simulink model "Task4_Simscape_model"  (R2026a)
settings: Solver=FixedStepAuto  StopTime=8  FixedStep=0.001
model workspace (MATLAB code in the model file):
  | clear; clc; close all;
values from neighbouring files (symbols this model uses):
  A0 = 0.310447780017169    (= 0.310447780017)    [Parameters.m]    (also in Parameters_optimization.m)
  B10 = -0.192075602039053    (= -0.192075602039)    [Parameters.m]    (also in Parameters_optimization.m)
  B20 = -0.011912003704451    (= -0.0119120037045)    [Parameters.m]    (also in Parameters_optimization.m)
  black = partTemplate    [Parameters.m]    (also in Parameters_optimization.m = struct)
  blueBlock = partTemplate    [Parameters.m]    (also in Parameters_optimization.m = struct)
  cyan = partTemplate    [Parameters.m]    (also in Parameters_optimization.m = struct)
  g = 9.81    [Parameters.m]    (also in Parameters_optimization.m)
  G0 = -1.061422531644424    (= -1.06142253164)    [Parameters.m]    (also in Parameters_optimization.m)
  greenBeam = partTemplate    [Parameters.m]    (also in Parameters_optimization.m = struct)
  greenBlock = partTemplate    [Parameters.m]    (also in Parameters_optimization.m = struct)
  grey = partTemplate    [Parameters.m]    (also in Parameters_optimization.m = struct)
  H0 = -0.357470264672538    (= -0.357470264673)    [Parameters.m]    (also in Parameters_optimization.m)
  I0 = -1.033155420835947    (= -1.03315542084)    [Parameters.m]    (also in Parameters_optimization.m)
  JM = 0.002    [Parameters.m]    (also in Parameters_optimization.m)
  LB1 = 0.8    [Parameters.m]    (also in Parameters_optimization.m)
  LB2 = 0.3    [Parameters.m]    (also in Parameters_optimization.m)
  LB3 = 0.24    [Parameters.m]    (also in Parameters_optimization.m)
  Lblack1 = 0.2    [Parameters.m]    (also in Parameters_optimization.m)
  LC1 = 0.4    [Parameters.m]    (also in Parameters_optimization.m)
  LC2 = 0.225    [Parameters.m]    (also in Parameters_optimization.m)
  LG1 = 0.3    [Parameters.m]    (also in Parameters_optimization.m)
  LG2 = 0.8    [Parameters.m]    (also in Parameters_optimization.m)
  Lgrey1 = 1.175    [Parameters.m]    (also in Parameters_optimization.m)
  lightBlue = partTemplate    [Parameters.m]    (also in Parameters_optimization.m = struct)
  LLB1 = 0.248    [Parameters.m]    (also in Parameters_optimization.m)
  LLB2 = 0.235    [Parameters.m]    (also in Parameters_optimization.m)
  LR1 = 1.05    [Parameters.m]    (also in Parameters_optimization.m)
  LW1 = 1.05    [Parameters.m]    (also in Parameters_optimization.m)
  nA = 200    [Parameters.m]    (also in Parameters_optimization.m = 100)
  nB1 = 200    [Parameters.m]    (also in Parameters_optimization.m = 100)
  nB2 = 200    [Parameters.m]    (also in Parameters_optimization.m)
  nG = 20    [Parameters.m]    (also in Parameters_optimization.m)
  nH = 100    [Parameters.m]    (also in Parameters_optimization.m = 50)
  nI = 20    [Parameters.m]    (also in Parameters_optimization.m)
  red = partTemplate    [Parameters.m]    (also in Parameters_optimization.m = struct)
  trajCoeff = coeff    [Parameters.m]    (also in Parameters_optimization.m = [2000 500 1600; Path_Planning_Robot.m)
  trajTime = t    [Parameters.m]    (also in Parameters_optimization.m = [0 2 4 6 8]; Path_Planning_Robot.m)
  w = 0.1    [Parameters.m]    (also in Parameters_optimization.m)
  white = partTemplate    [Parameters.m]    (also in Parameters_optimization.m = struct)
undefined symbols (not defined in the file or in its folder): X, Y, Z
libraries: sm_lib x152, nesl_utility x69, simulink x1
(part 2 of 5)

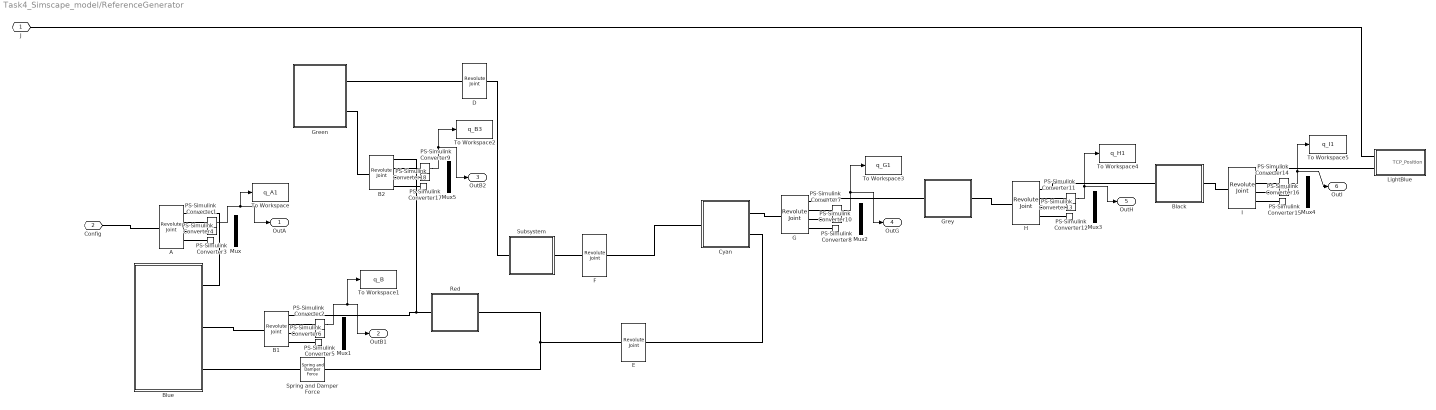
== system Task4_Simscape_model/ReferenceGenerator ==
  A : sm_lib/Joints/Revolute Joint  JointMode=Normal  CompositeWrenchDir=FollowerOnBase  CompositeWrenchFrame=BaseFrame  SenseConstraintForce=off  SenseConstraintTorque=off  SenseTotalForce=off  SenseTotalTorque=off  PositionTargetSpecify=off  PositionTargetPriority=High  PositionTargetValue=0  PositionTargetValueUnits=deg  VelocityTargetSpecify=off  VelocityTargetPriority=High  VelocityTargetValue=0  VelocityTargetValueUnits=deg/s  EquilibriumPosition=0  EquilibriumPositionUnits=deg  SpringStiffness=0  SpringStiffnessUnits=N*m/deg  DampingCoefficient=0  DampingCoefficientUnits=N*m/(deg/s)  LowerLimitSpecify=off  LowerLimitBound=-90  LowerLimitBoundUnits=deg  LowerLimitStiffness=1e4  LowerLimitStiffnessUnits=N*m/deg  LowerLimitDamping=10  LowerLimitDampingUnits=N*m/(deg/s)  LowerLimitTransitionRegionWidth=0.1  LowerLimitTransitionRegionWidthUnits=deg  UpperLimitSpecify=off  UpperLimitBound=90  UpperLimitBoundUnits=deg  UpperLimitStiffness=1e4  UpperLimitStiffnessUnits=N*m/deg  UpperLimitDamping=10  UpperLimitDampingUnits=N*m/(deg/s)  UpperLimitTransitionRegionWidth=0.1  UpperLimitTransitionRegionWidthUnits=deg  TorqueActuationMode=NoTorque  MotionActuationMode=ComputedMotion  SensePosition=on  SenseVelocity=on  SenseAcceleration=on  SenseTorqueForce=off  SenseLowerLimitTorqueForce=off  SenseUpperLimitTorqueForce=off
  B1 : sm_lib/Joints/Revolute Joint  JointMode=Normal  CompositeWrenchDir=FollowerOnBase  CompositeWrenchFrame=BaseFrame  SenseConstraintForce=off  SenseConstraintTorque=off  SenseTotalForce=off  SenseTotalTorque=off  PositionTargetSpecify=off  PositionTargetPriority=High  PositionTargetValue=0  PositionTargetValueUnits=deg  VelocityTargetSpecify=off  VelocityTargetPriority=High  VelocityTargetValue=0  VelocityTargetValueUnits=deg/s  EquilibriumPosition=0  EquilibriumPositionUnits=deg  SpringStiffness=0  SpringStiffnessUnits=N*m/deg  DampingCoefficient=0  DampingCoefficientUnits=N*m/(deg/s)  LowerLimitSpecify=on  LowerLimitBound=-80  LowerLimitBoundUnits=deg  LowerLimitStiffness=1e6  LowerLimitStiffnessUnits=N*m/deg  LowerLimitDamping=1000  LowerLimitDampingUnits=N*m/(deg/s)  LowerLimitTransitionRegionWidth=0.1  LowerLimitTransitionRegionWidthUnits=deg  UpperLimitSpecify=on  UpperLimitBound=80  UpperLimitBoundUnits=deg  UpperLimitStiffness=1e6  UpperLimitStiffnessUnits=N*m/deg  UpperLimitDamping=1000  UpperLimitDampingUnits=N*m/(deg/s)  UpperLimitTransitionRegionWidth=0.1  UpperLimitTransitionRegionWidthUnits=deg  TorqueActuationMode=NoTorque  MotionActuationMode=ComputedMotion  SensePosition=on  SenseVelocity=on  SenseAcceleration=on  SenseTorqueForce=off  SenseLowerLimitTorqueForce=off  SenseUpperLimitTorqueForce=off
  B2 : sm_lib/Joints/Revolute Joint  JointMode=Normal  CompositeWrenchDir=FollowerOnBase  CompositeWrenchFrame=BaseFrame  SenseConstraintForce=off  SenseConstraintTorque=off  SenseTotalForce=off  SenseTotalTorque=off  PositionTargetSpecify=off  PositionTargetPriority=High  PositionTargetValue=0  PositionTargetValueUnits=deg  VelocityTargetSpecify=off  VelocityTargetPriority=High  VelocityTargetValue=0  VelocityTargetValueUnits=deg/s  EquilibriumPosition=0  EquilibriumPositionUnits=deg  SpringStiffness=0  SpringStiffnessUnits=N*m/deg  DampingCoefficient=0  DampingCoefficientUnits=N*m/(deg/s)  LowerLimitSpecify=off  LowerLimitBound=-90  LowerLimitBoundUnits=deg  LowerLimitStiffness=1e4  LowerLimitStiffnessUnits=N*m/deg  LowerLimitDamping=10  LowerLimitDampingUnits=N*m/(deg/s)  LowerLimitTransitionRegionWidth=0.1  LowerLimitTransitionRegionWidthUnits=deg  UpperLimitSpecify=off  UpperLimitBound=90  UpperLimitBoundUnits=deg  UpperLimitStiffness=1e4  UpperLimitStiffnessUnits=N*m/deg  UpperLimitDamping=10  UpperLimitDampingUnits=N*m/(deg/s)  UpperLimitTransitionRegionWidth=0.1  UpperLimitTransitionRegionWidthUnits=deg  TorqueActuationMode=NoTorque  MotionActuationMode=ComputedMotion  SensePosition=on  SenseVelocity=on  SenseAcceleration=on  SenseTorqueForce=off  SenseLowerLimitTorqueForce=off  SenseUpperLimitTorqueForce=off
  Black : Subsystem
  Blue : Subsystem
  Cyan : Subsystem
  D : sm_lib/Joints/Revolute Joint  JointMode=Normal  CompositeWrenchDir=FollowerOnBase  CompositeWrenchFrame=BaseFrame  SenseConstraintForce=off  SenseConstraintTorque=off  SenseTotalForce=off  SenseTotalTorque=off  PositionTargetSpecify=off  PositionTargetPriority=High  PositionTargetValue=0  PositionTargetValueUnits=deg  VelocityTargetSpecify=off  VelocityTargetPriority=High  VelocityTargetValue=0  VelocityTargetValueUnits=deg/s  EquilibriumPosition=0  EquilibriumPositionUnits=deg  SpringStiffness=0  SpringStiffnessUnits=N*m/deg  DampingCoefficient=0  DampingCoefficientUnits=N*m/(deg/s)  LowerLimitSpecify=off  LowerLimitBound=-90  LowerLimitBoundUnits=deg  LowerLimitStiffness=1e4  LowerLimitStiffnessUnits=N*m/deg  LowerLimitDamping=10  LowerLimitDampingUnits=N*m/(deg/s)  LowerLimitTransitionRegionWidth=0.1  LowerLimitTransitionRegionWidthUnits=deg  UpperLimitSpecify=off  UpperLimitBound=90  UpperLimitBoundUnits=deg  UpperLimitStiffness=1e4  UpperLimitStiffnessUnits=N*m/deg  UpperLimitDamping=10  UpperLimitDampingUnits=N*m/(deg/s)  UpperLimitTransitionRegionWidth=0.1  UpperLimitTransitionRegionWidthUnits=deg  TorqueActuationMode=NoTorque  MotionActuationMode=ComputedMotion  SensePosition=off  SenseVelocity=off  SenseAcceleration=off  SenseTorqueForce=off  SenseLowerLimitTorqueForce=off  SenseUpperLimitTorqueForce=off
  E : sm_lib/Joints/Revolute Joint  JointMode=Normal  CompositeWrenchDir=FollowerOnBase  CompositeWrenchFrame=BaseFrame  SenseConstraintForce=off  SenseConstraintTorque=off  SenseTotalForce=off  SenseTotalTorque=off  PositionTargetSpecify=off  PositionTargetPriority=High  PositionTargetValue=0  PositionTargetValueUnits=deg  VelocityTargetSpecify=off  VelocityTargetPriority=High  VelocityTargetValue=0  VelocityTargetValueUnits=deg/s  EquilibriumPosition=0  EquilibriumPositionUnits=deg  SpringStiffness=0  SpringStiffnessUnits=N*m/deg  DampingCoefficient=0  DampingCoefficientUnits=N*m/(deg/s)  LowerLimitSpecify=on  LowerLimitBound=-80  LowerLimitBoundUnits=deg  LowerLimitStiffness=1e6  LowerLimitStiffnessUnits=N*m/deg  LowerLimitDamping=100000  LowerLimitDampingUnits=N*m/(deg/s)  LowerLimitTransitionRegionWidth=0.1  LowerLimitTransitionRegionWidthUnits=deg  UpperLimitSpecify=on  UpperLimitBound=80  UpperLimitBoundUnits=deg  UpperLimitStiffness=1e6  UpperLimitStiffnessUnits=N*m/deg  UpperLimitDamping=100000  UpperLimitDampingUnits=N*m/(deg/s)  UpperLimitTransitionRegionWidth=0.1  UpperLimitTransitionRegionWidthUnits=deg  TorqueActuationMode=NoTorque  MotionActuationMode=ComputedMotion  SensePosition=off  SenseVelocity=off  SenseAcceleration=off  SenseTorqueForce=off  SenseLowerLimitTorqueForce=off  SenseUpperLimitTorqueForce=off
  F : sm_lib/Joints/Revolute Joint  JointMode=Normal  CompositeWrenchDir=FollowerOnBase  CompositeWrenchFrame=BaseFrame  SenseConstraintForce=off  SenseConstraintTorque=off  SenseTotalForce=off  SenseTotalTorque=off  PositionTargetSpecify=off  PositionTargetPriority=High  PositionTargetValue=0  PositionTargetValueUnits=deg  VelocityTargetSpecify=off  VelocityTargetPriority=High  VelocityTargetValue=0  VelocityTargetValueUnits=deg/s  EquilibriumPosition=0  EquilibriumPositionUnits=deg  SpringStiffness=0  SpringStiffnessUnits=N*m/deg  DampingCoefficient=0  DampingCoefficientUnits=N*m/(deg/s)  LowerLimitSpecify=off  LowerLimitBound=-90  LowerLimitBoundUnits=deg  LowerLimitStiffness=1e4  LowerLimitStiffnessUnits=N*m/deg  LowerLimitDamping=10  LowerLimitDampingUnits=N*m/(deg/s)  LowerLimitTransitionRegionWidth=0.1  LowerLimitTransitionRegionWidthUnits=deg  UpperLimitSpecify=off  UpperLimitBound=90  UpperLimitBoundUnits=deg  UpperLimitStiffness=1e4  UpperLimitStiffnessUnits=N*m/deg  UpperLimitDamping=10  UpperLimitDampingUnits=N*m/(deg/s)  UpperLimitTransitionRegionWidth=0.1  UpperLimitTransitionRegionWidthUnits=deg  TorqueActuationMode=NoTorque  MotionActuationMode=ComputedMotion  SensePosition=off  SenseVelocity=off  SenseAcceleration=off  SenseTorqueForce=off  SenseLowerLimitTorqueForce=off  SenseUpperLimitTorqueForce=off
  G : sm_lib/Joints/Revolute Joint  JointMode=Normal  CompositeWrenchDir=FollowerOnBase  CompositeWrenchFrame=BaseFrame  SenseConstraintForce=off  SenseConstraintTorque=off  SenseTotalForce=off  SenseTotalTorque=off  PositionTargetSpecify=off  PositionTargetPriority=High  PositionTargetValue=0  PositionTargetValueUnits=deg  VelocityTargetSpecify=off  VelocityTargetPriority=High  VelocityTargetValue=0  VelocityTargetValueUnits=deg/s  EquilibriumPosition=0  EquilibriumPositionUnits=deg  SpringStiffness=0  SpringStiffnessUnits=N*m/deg  DampingCoefficient=0  DampingCoefficientUnits=N*m/(deg/s)  LowerLimitSpecify=off  LowerLimitBound=-90  LowerLimitBoundUnits=deg  LowerLimitStiffness=1e4  LowerLimitStiffnessUnits=N*m/deg  LowerLimitDamping=10  LowerLimitDampingUnits=N*m/(deg/s)  LowerLimitTransitionRegionWidth=0.1  LowerLimitTransitionRegionWidthUnits=deg  UpperLimitSpecify=off  UpperLimitBound=90  UpperLimitBoundUnits=deg  UpperLimitStiffness=1e4  UpperLimitStiffnessUnits=N*m/deg  UpperLimitDamping=10  UpperLimitDampingUnits=N*m/(deg/s)  UpperLimitTransitionRegionWidth=0.1  UpperLimitTransitionRegionWidthUnits=deg  TorqueActuationMode=NoTorque  MotionActuationMode=ComputedMotion  SensePosition=on  SenseVelocity=on  SenseAcceleration=on  SenseTorqueForce=off  SenseLowerLimitTorqueForce=off  SenseUpperLimitTorqueForce=off
  Green : Subsystem
  Grey : Subsystem
  H : sm_lib/Joints/Revolute Joint  JointMode=Normal  CompositeWrenchDir=FollowerOnBase  CompositeWrenchFrame=BaseFrame  SenseConstraintForce=off  SenseConstraintTorque=off  SenseTotalForce=off  SenseTotalTorque=off  PositionTargetSpecify=off  PositionTargetPriority=High  PositionTargetValue=0  PositionTargetValueUnits=deg  VelocityTargetSpecify=off  VelocityTargetPriority=High  VelocityTargetValue=0  VelocityTargetValueUnits=deg/s  EquilibriumPosition=0  EquilibriumPositionUnits=deg  SpringStiffness=0  SpringStiffnessUnits=N*m/deg  DampingCoefficient=0  DampingCoefficientUnits=N*m/(deg/s)  LowerLimitSpecify=on  LowerLimitBound=-90  LowerLimitBoundUnits=deg  LowerLimitStiffness=1e4  LowerLimitStiffnessUnits=N*m/deg  LowerLimitDamping=10  LowerLimitDampingUnits=N*m/(deg/s)  LowerLimitTransitionRegionWidth=0.1  LowerLimitTransitionRegionWidthUnits=deg  UpperLimitSpecify=on  UpperLimitBound=90  UpperLimitBoundUnits=deg  UpperLimitStiffness=1e4  UpperLimitStiffnessUnits=N*m/deg  UpperLimitDamping=10  UpperLimitDampingUnits=N*m/(deg/s)  UpperLimitTransitionRegionWidth=0.1  UpperLimitTransitionRegionWidthUnits=deg  TorqueActuationMode=NoTorque  MotionActuationMode=ComputedMotion  SensePosition=on  SenseVelocity=on  SenseAcceleration=on  SenseTorqueForce=off  SenseLowerLimitTorqueForce=off  SenseUpperLimitTorqueForce=off
  I : sm_lib/Joints/Revolute Joint  JointMode=Normal  CompositeWrenchDir=FollowerOnBase  CompositeWrenchFrame=BaseFrame  SenseConstraintForce=off  SenseConstraintTorque=off  SenseTotalForce=off  SenseTotalTorque=off  PositionTargetSpecify=off  PositionTargetPriority=High  PositionTargetValue=0  PositionTargetValueUnits=deg  VelocityTargetSpecify=off  VelocityTargetPriority=High  VelocityTargetValue=0  VelocityTargetValueUnits=deg/s  EquilibriumPosition=0  EquilibriumPositionUnits=deg  SpringStiffness=0  SpringStiffnessUnits=N*m/deg  DampingCoefficient=0  DampingCoefficientUnits=N*m/(deg/s)  LowerLimitSpecify=off  LowerLimitBound=-90  LowerLimitBoundUnits=deg  LowerLimitStiffness=1e4  LowerLimitStiffnessUnits=N*m/deg  LowerLimitDamping=10  LowerLimitDampingUnits=N*m/(deg/s)  LowerLimitTransitionRegionWidth=0.1  LowerLimitTransitionRegionWidthUnits=deg  UpperLimitSpecify=off  UpperLimitBound=90  UpperLimitBoundUnits=deg  UpperLimitStiffness=1e4  UpperLimitStiffnessUnits=N*m/deg  UpperLimitDamping=10  UpperLimitDampingUnits=N*m/(deg/s)  UpperLimitTransitionRegionWidth=0.1  UpperLimitTransitionRegionWidthUnits=deg  TorqueActuationMode=NoTorque  MotionActuationMode=ComputedMotion  SensePosition=on  SenseVelocity=on  SenseAcceleration=on  SenseTorqueForce=off  SenseLowerLimitTorqueForce=off  SenseUpperLimitTorqueForce=off
  LightBlue : Subsystem
  Mux{,1..5} (6 alike) : Mux  Inputs=3
  PS-Simulink Converter{1..18} (18 alike) : nesl_utility/PS-Simulink Converter  PhysicalDomain=network_engine_domain  SubClassName=ps_output  LeftPortType=input  RightPortType=output  PseudoPeriodic=off  Frequencies=[]  VectorFormat=inherit  Unit=inherit  AffineConversion=off
  Red : Subsystem
  Spring and Damper Force : sm_lib/Forces and Torques/Spring and Damper Force  NaturalLength=L0_spring  NaturalLengthUnits=m  SpringStiffness=k_spring  SpringStiffnessUnits=N/m  DampingCoefficient=0  DampingCoefficientUnits=N/(m/s)  SenseForce=off
  Subsystem : Subsystem
  To Workspace : ToWorkspace  VariableName=q_A1  SaveFormat=Timeseries  SampleTime=-1
  To Workspace1 : ToWorkspace  VariableName=q_B  SaveFormat=Timeseries  SampleTime=-1
  To Workspace2 : ToWorkspace  VariableName=q_B3  SaveFormat=Timeseries  SampleTime=-1
  To Workspace3 : ToWorkspace  VariableName=q_G1  SaveFormat=Timeseries  SampleTime=-1
  To Workspace4 : ToWorkspace  VariableName=q_H1  SaveFormat=Timeseries  SampleTime=-1
  To Workspace5 : ToWorkspace  VariableName=q_I1  SaveFormat=Timeseries  SampleTime=-1
  J : PMIOPort  Side=Left
  Config : PMIOPort  Port=2  Side=Left
  OutA : Outport
  OutB1 : Outport  Port=2
  OutB2 : Outport  Port=3
  OutG : Outport  Port=4
  OutH : Outport  Port=5
  OutI : Outport  Port=6
  wires:
  PS-Simulink Converter2/1 -> To Workspace1/1, OutB1/1
  PS-Simulink Converter1/1 -> To Workspace/1, OutA/1
  PS-Simulink Converter9/1 -> To Workspace2/1, OutB2/1
  PS-Simulink Converter7/1 -> To Workspace3/1, OutG/1
  PS-Simulink Converter11/1 -> To Workspace4/1, OutH/1
  PS-Simulink Converter14/1 -> To Workspace5/1, OutI/1
  connections:
  B2/RConn1 -- B1/RConn1 -- Red/RConn1
  LightBlue/LConn2 -- I/RConn1
  G/LConn1 -- Cyan/RConn1
  Spring and Damper Force/RConn1 -- Red/LConn1 -- E/LConn1
  Black/LConn1 -- H/RConn1
  F/LConn1 -- Subsystem/LConn1
  Spring and Damper Force/LConn1 -- Blue/RConn3
  Subsystem/RConn1 -- D/RConn1
  Green/RConn2 -- B2/LConn1
  I/LConn1 -- Black/RConn1
  A/LConn1 -- Config/RConn1
  Blue/RConn2 -- B1/LConn1
  H/LConn1 -- Grey/RConn1
  F/RConn1 -- Cyan/LConn1
  D/LConn1 -- Green/RConn1
  Grey/LConn1 -- G/RConn1
  Blue/RConn1 -- A/RConn1
  Cyan/RConn2 -- E/RConn1
  J/RConn1 -- LightBlue/LConn1
  PS-Simulink Converter1/LConn1 -- A/RConn2
  PS-Simulink Converter3/LConn1 -- A/RConn3
  PS-Simulink Converter4/LConn1 -- A/RConn4
  PS-Simulink Converter2/LConn1 -- B1/RConn2
  B1/RConn3 -- PS-Simulink Converter5/LConn1
  PS-Simulink Converter6/LConn1 -- B1/RConn4
  PS-Simulink Converter7/LConn1 -- G/RConn2
  G/RConn3 -- PS-Simulink Converter8/LConn1
  PS-Simulink Converter10/LConn1 -- G/RConn4
  PS-Simulink Converter11/LConn1 -- H/RConn2
  PS-Simulink Converter12/LConn1 -- H/RConn3
  PS-Simulink Converter13/LConn1 -- H/RConn4
  PS-Simulink Converter14/LConn1 -- I/RConn2
  PS-Simulink Converter15/LConn1 -- I/RConn3
  PS-Simulink Converter16/LConn1 -- I/RConn4
  PS-Simulink Converter9/LConn1 -- B2/RConn2
  PS-Simulink Converter17/LConn1 -- B2/RConn3
  PS-Simulink Converter18/LConn1 -- B2/RConn4

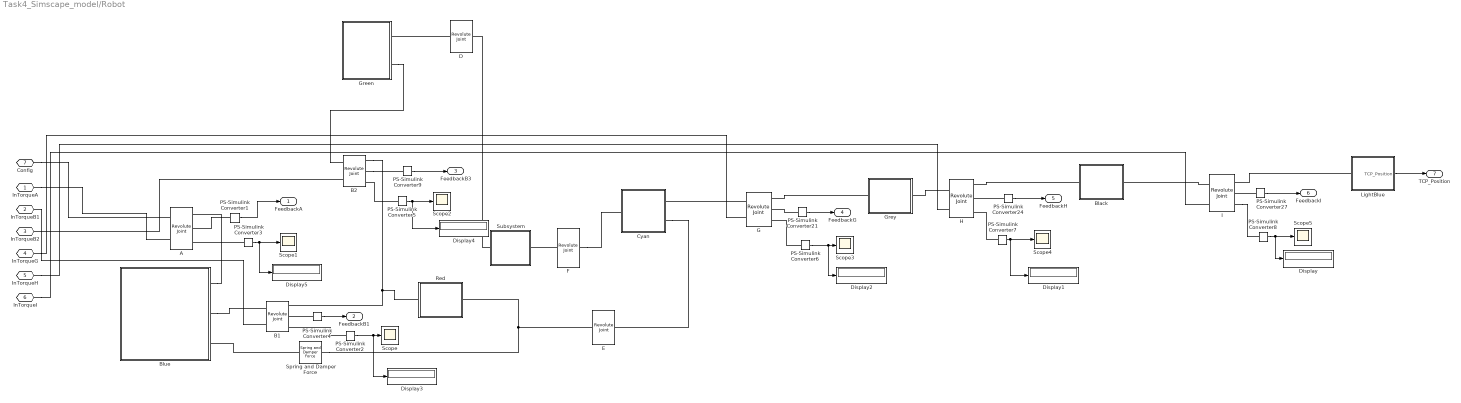
== system Task4_Simscape_model/Robot ==
  A : sm_lib/Joints/Revolute Joint  JointMode=Normal  CompositeWrenchDir=FollowerOnBase  CompositeWrenchFrame=BaseFrame  SenseConstraintForce=off  SenseConstraintTorque=off  SenseTotalForce=off  SenseTotalTorque=off  PositionTargetSpecify=on  PositionTargetPriority=High  PositionTargetValue=A0  PositionTargetValueUnits=rad  VelocityTargetSpecify=on  VelocityTargetPriority=High  VelocityTargetValue=0  VelocityTargetValueUnits=rad/s  EquilibriumPosition=0  EquilibriumPositionUnits=deg  SpringStiffness=0  SpringStiffnessUnits=N*m/deg  DampingCoefficient=0  DampingCoefficientUnits=N*m/(deg/s)  LowerLimitSpecify=off  LowerLimitBound=-90  LowerLimitBoundUnits=deg  LowerLimitStiffness=1e4  LowerLimitStiffnessUnits=N*m/deg  LowerLimitDamping=10  LowerLimitDampingUnits=N*m/(deg/s)  LowerLimitTransitionRegionWidth=0.1  LowerLimitTransitionRegionWidthUnits=deg  UpperLimitSpecify=off  UpperLimitBound=90  UpperLimitBoundUnits=deg  UpperLimitStiffness=1e4  UpperLimitStiffnessUnits=N*m/deg  UpperLimitDamping=10  UpperLimitDampingUnits=N*m/(deg/s)  UpperLimitTransitionRegionWidth=0.1  UpperLimitTransitionRegionWidthUnits=deg  TorqueActuationMode=InputTorque  MotionActuationMode=ComputedMotion  SensePosition=on  SenseVelocity=off  SenseAcceleration=off  SenseTorqueForce=on  SenseLowerLimitTorqueForce=off  SenseUpperLimitTorqueForce=off
  B1 : sm_lib/Joints/Revolute Joint  JointMode=Normal  CompositeWrenchDir=FollowerOnBase  CompositeWrenchFrame=BaseFrame  SenseConstraintForce=off  SenseConstraintTorque=off  SenseTotalForce=off  SenseTotalTorque=off  PositionTargetSpecify=on  PositionTargetPriority=High  PositionTargetValue=B10  PositionTargetValueUnits=rad  VelocityTargetSpecify=on  VelocityTargetPriority=High  VelocityTargetValue=0  VelocityTargetValueUnits=rad/s  EquilibriumPosition=0  EquilibriumPositionUnits=deg  SpringStiffness=0  SpringStiffnessUnits=N*m/deg  DampingCoefficient=0  DampingCoefficientUnits=N*m/(deg/s)  LowerLimitSpecify=on  LowerLimitBound=-80  LowerLimitBoundUnits=deg  LowerLimitStiffness=1000  LowerLimitStiffnessUnits=N*m/deg  LowerLimitDamping=1000  LowerLimitDampingUnits=N*m/(deg/s)  LowerLimitTransitionRegionWidth=0.1  LowerLimitTransitionRegionWidthUnits=deg  UpperLimitSpecify=on  UpperLimitBound=80  UpperLimitBoundUnits=deg  UpperLimitStiffness=1000  UpperLimitStiffnessUnits=N*m/deg  UpperLimitDamping=1000  UpperLimitDampingUnits=N*m/(deg/s)  UpperLimitTransitionRegionWidth=0.1  UpperLimitTransitionRegionWidthUnits=deg  TorqueActuationMode=InputTorque  MotionActuationMode=ComputedMotion  SensePosition=on  SenseVelocity=off  SenseAcceleration=off  SenseTorqueForce=on  SenseLowerLimitTorqueForce=off  SenseUpperLimitTorqueForce=off
  B2 : sm_lib/Joints/Revolute Joint  JointMode=Normal  CompositeWrenchDir=FollowerOnBase  CompositeWrenchFrame=BaseFrame  SenseConstraintForce=off  SenseConstraintTorque=off  SenseTotalForce=off  SenseTotalTorque=off  PositionTargetSpecify=on  PositionTargetPriority=High  PositionTargetValue=B20  PositionTargetValueUnits=rad  VelocityTargetSpecify=on  VelocityTargetPriority=High  VelocityTargetValue=0  VelocityTargetValueUnits=rad/s  EquilibriumPosition=0  EquilibriumPositionUnits=deg  SpringStiffness=0  SpringStiffnessUnits=N*m/deg  DampingCoefficient=0  DampingCoefficientUnits=N*m/(deg/s)  LowerLimitSpecify=off  LowerLimitBound=-90  LowerLimitBoundUnits=deg  LowerLimitStiffness=1e4  LowerLimitStiffnessUnits=N*m/deg  LowerLimitDamping=10  LowerLimitDampingUnits=N*m/(deg/s)  LowerLimitTransitionRegionWidth=0.1  LowerLimitTransitionRegionWidthUnits=deg  UpperLimitSpecify=off  UpperLimitBound=90  UpperLimitBoundUnits=deg  UpperLimitStiffness=1e4  UpperLimitStiffnessUnits=N*m/deg  UpperLimitDamping=10  UpperLimitDampingUnits=N*m/(deg/s)  UpperLimitTransitionRegionWidth=0.1  UpperLimitTransitionRegionWidthUnits=deg  TorqueActuationMode=InputTorque  MotionActuationMode=ComputedMotion  SensePosition=on  SenseVelocity=off  SenseAcceleration=off  SenseTorqueForce=on  SenseLowerLimitTorqueForce=off  SenseUpperLimitTorqueForce=off
  Black : Subsystem
  Blue : Subsystem
  Cyan : Subsystem
  D : sm_lib/Joints/Revolute Joint  JointMode=Normal  CompositeWrenchDir=FollowerOnBase  CompositeWrenchFrame=BaseFrame  SenseConstraintForce=off  SenseConstraintTorque=off  SenseTotalForce=off  SenseTotalTorque=off  PositionTargetSpecify=off  PositionTargetPriority=High  PositionTargetValue=0  PositionTargetValueUnits=deg  VelocityTargetSpecify=off  VelocityTargetPriority=High  VelocityTargetValue=0  VelocityTargetValueUnits=deg/s  EquilibriumPosition=0  EquilibriumPositionUnits=deg  SpringStiffness=0  SpringStiffnessUnits=N*m/deg  DampingCoefficient=0  DampingCoefficientUnits=N*m/(deg/s)  LowerLimitSpecify=off  LowerLimitBound=-90  LowerLimitBoundUnits=deg  LowerLimitStiffness=1e4  LowerLimitStiffnessUnits=N*m/deg  LowerLimitDamping=10  LowerLimitDampingUnits=N*m/(deg/s)  LowerLimitTransitionRegionWidth=0.1  LowerLimitTransitionRegionWidthUnits=deg  UpperLimitSpecify=off  UpperLimitBound=90  UpperLimitBoundUnits=deg  UpperLimitStiffness=1e4  UpperLimitStiffnessUnits=N*m/deg  UpperLimitDamping=10  UpperLimitDampingUnits=N*m/(deg/s)  UpperLimitTransitionRegionWidth=0.1  UpperLimitTransitionRegionWidthUnits=deg  TorqueActuationMode=NoTorque  MotionActuationMode=ComputedMotion  SensePosition=off  SenseVelocity=off  SenseAcceleration=off  SenseTorqueForce=off  SenseLowerLimitTorqueForce=off  SenseUpperLimitTorqueForce=off
  Display{,1..5} (6 alike) : Display
  E : sm_lib/Joints/Revolute Joint  JointMode=Normal  CompositeWrenchDir=FollowerOnBase  CompositeWrenchFrame=BaseFrame  SenseConstraintForce=off  SenseConstraintTorque=off  SenseTotalForce=off  SenseTotalTorque=off  PositionTargetSpecify=off  PositionTargetPriority=High  PositionTargetValue=0  PositionTargetValueUnits=deg  VelocityTargetSpecify=off  VelocityTargetPriority=High  VelocityTargetValue=0  VelocityTargetValueUnits=deg/s  EquilibriumPosition=0  EquilibriumPositionUnits=deg  SpringStiffness=0  SpringStiffnessUnits=N*m/deg  DampingCoefficient=0  DampingCoefficientUnits=N*m/(deg/s)  LowerLimitSpecify=on  LowerLimitBound=-80  LowerLimitBoundUnits=deg  LowerLimitStiffness=1e6  LowerLimitStiffnessUnits=N*m/deg  LowerLimitDamping=100000  LowerLimitDampingUnits=N*m/(deg/s)  LowerLimitTransitionRegionWidth=0.1  LowerLimitTransitionRegionWidthUnits=deg  UpperLimitSpecify=on  UpperLimitBound=80  UpperLimitBoundUnits=deg  UpperLimitStiffness=1e6  UpperLimitStiffnessUnits=N*m/deg  UpperLimitDamping=100000  UpperLimitDampingUnits=N*m/(deg/s)  UpperLimitTransitionRegionWidth=0.1  UpperLimitTransitionRegionWidthUnits=deg  TorqueActuationMode=NoTorque  MotionActuationMode=ComputedMotion  SensePosition=off  SenseVelocity=off  SenseAcceleration=off  SenseTorqueForce=off  SenseLowerLimitTorqueForce=off  SenseUpperLimitTorqueForce=off
  F : sm_lib/Joints/Revolute Joint  JointMode=Normal  CompositeWrenchDir=FollowerOnBase  CompositeWrenchFrame=BaseFrame  SenseConstraintForce=off  SenseConstraintTorque=off  SenseTotalForce=off  SenseTotalTorque=off  PositionTargetSpecify=off  PositionTargetPriority=High  PositionTargetValue=0  PositionTargetValueUnits=deg  VelocityTargetSpecify=off  VelocityTargetPriority=High  VelocityTargetValue=0  VelocityTargetValueUnits=deg/s  EquilibriumPosition=0  EquilibriumPositionUnits=deg  SpringStiffness=0  SpringStiffnessUnits=N*m/deg  DampingCoefficient=0  DampingCoefficientUnits=N*m/(deg/s)  LowerLimitSpecify=off  LowerLimitBound=-90  LowerLimitBoundUnits=deg  LowerLimitStiffness=1e4  LowerLimitStiffnessUnits=N*m/deg  LowerLimitDamping=10  LowerLimitDampingUnits=N*m/(deg/s)  LowerLimitTransitionRegionWidth=0.1  LowerLimitTransitionRegionWidthUnits=deg  UpperLimitSpecify=off  UpperLimitBound=90  UpperLimitBoundUnits=deg  UpperLimitStiffness=1e4  UpperLimitStiffnessUnits=N*m/deg  UpperLimitDamping=10  UpperLimitDampingUnits=N*m/(deg/s)  UpperLimitTransitionRegionWidth=0.1  UpperLimitTransitionRegionWidthUnits=deg  TorqueActuationMode=NoTorque  MotionActuationMode=ComputedMotion  SensePosition=off  SenseVelocity=off  SenseAcceleration=off  SenseTorqueForce=off  SenseLowerLimitTorqueForce=off  SenseUpperLimitTorqueForce=off
  G : sm_lib/Joints/Revolute Joint  JointMode=Normal  CompositeWrenchDir=FollowerOnBase  CompositeWrenchFrame=BaseFrame  SenseConstraintForce=off  SenseConstraintTorque=off  SenseTotalForce=off  SenseTotalTorque=off  PositionTargetSpecify=on  PositionTargetPriority=High  PositionTargetValue=G0  PositionTargetValueUnits=rad  VelocityTargetSpecify=on  VelocityTargetPriority=High  VelocityTargetValue=0  VelocityTargetValueUnits=rad/s  EquilibriumPosition=0  EquilibriumPositionUnits=deg  SpringStiffness=0  SpringStiffnessUnits=N*m/deg  DampingCoefficient=0  DampingCoefficientUnits=N*m/(deg/s)  LowerLimitSpecify=off  LowerLimitBound=-90  LowerLimitBoundUnits=deg  LowerLimitStiffness=1e4  LowerLimitStiffnessUnits=N*m/deg  LowerLimitDamping=10  LowerLimitDampingUnits=N*m/(deg/s)  LowerLimitTransitionRegionWidth=0.1  LowerLimitTransitionRegionWidthUnits=deg  UpperLimitSpecify=off  UpperLimitBound=90  UpperLimitBoundUnits=deg  UpperLimitStiffness=1e4  UpperLimitStiffnessUnits=N*m/deg  UpperLimitDamping=10  UpperLimitDampingUnits=N*m/(deg/s)  UpperLimitTransitionRegionWidth=0.1  UpperLimitTransitionRegionWidthUnits=deg  TorqueActuationMode=InputTorque  MotionActuationMode=ComputedMotion  SensePosition=on  SenseVelocity=off  SenseAcceleration=off  SenseTorqueForce=on  SenseLowerLimitTorqueForce=off  SenseUpperLimitTorqueForce=off
  Green : Subsystem
  Grey : Subsystem
  H : sm_lib/Joints/Revolute Joint  JointMode=Normal  CompositeWrenchDir=FollowerOnBase  CompositeWrenchFrame=BaseFrame  SenseConstraintForce=off  SenseConstraintTorque=off  SenseTotalForce=off  SenseTotalTorque=off  PositionTargetSpecify=on  PositionTargetPriority=High  PositionTargetValue=H0  PositionTargetValueUnits=rad  VelocityTargetSpecify=on  VelocityTargetPriority=High  VelocityTargetValue=0  VelocityTargetValueUnits=rad/s  EquilibriumPosition=0  EquilibriumPositionUnits=deg  SpringStiffness=0  SpringStiffnessUnits=N*m/deg  DampingCoefficient=0  DampingCoefficientUnits=N*m/(deg/s)  LowerLimitSpecify=off  LowerLimitBound=-90  LowerLimitBoundUnits=deg  LowerLimitStiffness=100  LowerLimitStiffnessUnits=N*m/deg  LowerLimitDamping=1000  LowerLimitDampingUnits=N*m/(deg/s)  LowerLimitTransitionRegionWidth=0.1  LowerLimitTransitionRegionWidthUnits=deg  UpperLimitSpecify=off  UpperLimitBound=90  UpperLimitBoundUnits=deg  UpperLimitStiffness=100  UpperLimitStiffnessUnits=N*m/deg  UpperLimitDamping=1000  UpperLimitDampingUnits=N*m/(deg/s)  UpperLimitTransitionRegionWidth=0.1  UpperLimitTransitionRegionWidthUnits=deg  TorqueActuationMode=InputTorque  MotionActuationMode=ComputedMotion  SensePosition=on  SenseVelocity=off  SenseAcceleration=off  SenseTorqueForce=on  SenseLowerLimitTorqueForce=off  SenseUpperLimitTorqueForce=off
  I : sm_lib/Joints/Revolute Joint  JointMode=Normal  CompositeWrenchDir=FollowerOnBase  CompositeWrenchFrame=BaseFrame  SenseConstraintForce=off  SenseConstraintTorque=off  SenseTotalForce=off  SenseTotalTorque=off  PositionTargetSpecify=on  PositionTargetPriority=High  PositionTargetValue=I0  PositionTargetValueUnits=rad  VelocityTargetSpecify=on  VelocityTargetPriority=High  VelocityTargetValue=0  VelocityTargetValueUnits=rad/s  EquilibriumPosition=0  EquilibriumPositionUnits=deg  SpringStiffness=0  SpringStiffnessUnits=N*m/deg  DampingCoefficient=0  DampingCoefficientUnits=N*m/(deg/s)  LowerLimitSpecify=on  LowerLimitBound=-90  LowerLimitBoundUnits=deg  LowerLimitStiffness=1e5  LowerLimitStiffnessUnits=N*m/deg  LowerLimitDamping=100  LowerLimitDampingUnits=N*m/(deg/s)  LowerLimitTransitionRegionWidth=0.1  LowerLimitTransitionRegionWidthUnits=deg  UpperLimitSpecify=on  UpperLimitBound=90  UpperLimitBoundUnits=deg  UpperLimitStiffness=1e5  UpperLimitStiffnessUnits=N*m/deg  UpperLimitDamping=100  UpperLimitDampingUnits=N*m/(deg/s)  UpperLimitTransitionRegionWidth=0.1  UpperLimitTransitionRegionWidthUnits=deg  TorqueActuationMode=InputTorque  MotionActuationMode=ComputedMotion  SensePosition=on  SenseVelocity=off  SenseAcceleration=off  SenseTorqueForce=on  SenseLowerLimitTorqueForce=off  SenseUpperLimitTorqueForce=off
  LightBlue : Subsystem
  PS-Simulink Converter{1..9,21,24,27} (12 alike) : nesl_utility/PS-Simulink Converter  PhysicalDomain=network_engine_domain  SubClassName=ps_output  LeftPortType=input  RightPortType=output  PseudoPeriodic=off  Frequencies=[]  VectorFormat=inherit  Unit=inherit  AffineConversion=off
  Red : Subsystem
  Scope{,1..5} (6 alike) : Scope
      Scope settings: ActiveDisplayYMinimum=-1183.9928415101156  ActiveDisplayYMaximum=-1183.9928415101133  DataLoggingVariableName=ScopeData10
      Scope1 settings: ActiveDisplayYMinimum=-1  ActiveDisplayYMaximum=1  DataLoggingVariableName=ScopeData11
      Scope2 settings: ActiveDisplayYMinimum=-1  ActiveDisplayYMaximum=1  DataLoggingVariableName=ScopeData12
      Scope3 settings: ActiveDisplayYMinimum=76.287342511896966  ActiveDisplayYMaximum=76.2873425118971  DataLoggingVariableName=ScopeData13
      Scope4 settings: ActiveDisplayYMinimum=-1  ActiveDisplayYMaximum=1  DataLoggingVariableName=ScopeData14
      Scope5 settings: ActiveDisplayYMinimum=-1  ActiveDisplayYMaximum=1  DataLoggingVariableName=ScopeData15
  Spring and Damper Force : sm_lib/Forces and Torques/Spring and Damper Force  NaturalLength=L0_spring  NaturalLengthUnits=m  SpringStiffness=k_spring  SpringStiffnessUnits=N/m  DampingCoefficient=0  DampingCoefficientUnits=N/(m/s)  SenseForce=off
  Subsystem : Subsystem
  InTorqueA : PMIOPort  Side=Left
  InTorqueB1 : PMIOPort  Port=2  Side=Left
  InTorqueB2 : PMIOPort  Port=3  Side=Left
  InTorqueG : PMIOPort  Port=4  Side=Left
  InTorqueH : PMIOPort  Port=5  Side=Left
  InTorqueI : PMIOPort  Port=6  Side=Left
  Config : PMIOPort  Port=7  Side=Left
  FeedbackA : Outport
  FeedbackB1 : Outport  Port=2
  FeedbackB3 : Outport  Port=3
  FeedbackG : Outport  Port=4
  FeedbackH : Outport  Port=5
  FeedbackI : Outport  Port=6
  TCP_Position : Outport  Port=7
  wires:
  PS-Simulink Converter1/1 -> FeedbackA/1
  PS-Simulink Converter4/1 -> FeedbackB1/1
  PS-Simulink Converter9/1 -> FeedbackB3/1
  LightBlue/1(TCP_Position) -> TCP_Position/1
  PS-Simulink Converter21/1 -> FeedbackG/1
  PS-Simulink Converter27/1 -> FeedbackI/1
  PS-Simulink Converter24/1 -> FeedbackH/1
  PS-Simulink Converter2/1 -> Display3/1, Scope/1
  PS-Simulink Converter3/1 -> Display5/1, Scope1/1
  PS-Simulink Converter5/1 -> Display4/1, Scope2/1
  PS-Simulink Converter6/1 -> Display2/1, Scope3/1
  PS-Simulink Converter7/1 -> Display1/1, Scope4/1
  PS-Simulink Converter8/1 -> Display/1, Scope5/1
  connections:
  B2/RConn1 -- Red/RConn1 -- B1/RConn1
  LightBlue/LConn1 -- I/RConn1
  G/LConn1 -- Cyan/RConn1
  Spring and Damper Force/RConn1 -- E/LConn1 -- Red/LConn1
  Black/LConn1 -- H/RConn1
  F/LConn1 -- Subsystem/LConn1
  Spring and Damper Force/LConn1 -- Blue/RConn3
  Subsystem/RConn1 -- D/RConn1
  Green/RConn2 -- B2/LConn1
  I/LConn1 -- Black/RConn1
  Blue/RConn2 -- B1/LConn1
  PS-Simulink Converter1/LConn1 -- A/RConn2
  PS-Simulink Converter27/LConn1 -- I/RConn2
  H/LConn1 -- Grey/RConn1
  F/RConn1 -- Cyan/LConn1
  D/LConn1 -- Green/RConn1
  Grey/LConn1 -- G/RConn1
  Blue/RConn1 -- A/RConn1
  Cyan/RConn2 -- E/RConn1
  PS-Simulink Converter21/LConn1 -- G/RConn2
  B2/RConn2 -- PS-Simulink Converter9/LConn1
  PS-Simulink Converter4/LConn1 -- B1/RConn2
  PS-Simulink Converter24/LConn1 -- H/RConn2
  Config/RConn1 -- A/LConn1
  PS-Simulink Converter2/LConn1 -- B1/RConn3
  PS-Simulink Converter3/LConn1 -- A/RConn3
  PS-Simulink Converter5/LConn1 -- B2/RConn3
  PS-Simulink Converter6/LConn1 -- G/RConn3
  PS-Simulink Converter7/LConn1 -- H/RConn3
  I/RConn3 -- PS-Simulink Converter8/LConn1
  InTorqueA/RConn1 -- A/LConn2
  B2/LConn2 -- InTorqueB2/RConn1
  InTorqueG/RConn1 -- G/LConn2
  InTorqueH/RConn1 -- H/LConn2
  InTorqueI/RConn1 -- I/LConn2
  InTorqueB1/RConn1 -- B1/LConn2

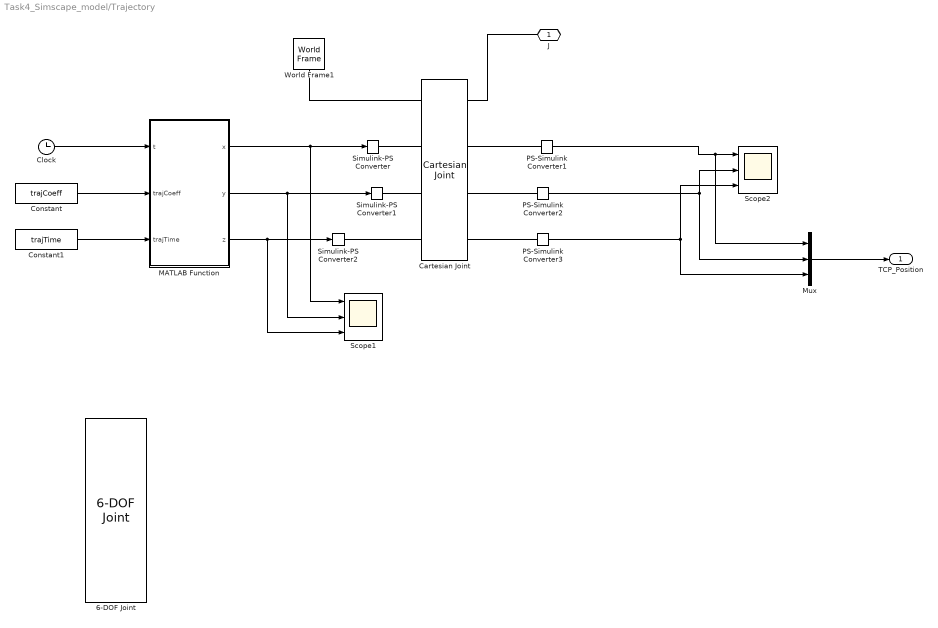
== system Task4_Simscape_model/Trajectory ==
  6-DOF Joint : sm_lib/Joints/6-DOF Joint  JointMode=Normal  CompositeWrenchDir=FollowerOnBase  CompositeWrenchFrame=BaseFrame  SenseConstraintForce=off  SenseConstraintTorque=off  SenseTotalForce=off  SenseTotalTorque=off  PxPositionTargetSpecify=off  PxPositionTargetPriority=High  PxPositionTargetValue=0  PxPositionTargetValueUnits=m  PxVelocityTargetSpecify=off  PxVelocityTargetPriority=High  PxVelocityTargetValue=0  PxVelocityTargetValueUnits=m/s  PxEquilibriumPosition=0  PxEquilibriumPositionUnits=m  PxSpringStiffness=0  PxSpringStiffnessUnits=N/m  PxDampingCoefficient=0  PxDampingCoefficientUnits=N/(m/s)  PxLowerLimitSpecify=off  PxLowerLimitBound=-1  PxLowerLimitBoundUnits=m  PxLowerLimitStiffness=1e6  PxLowerLimitStiffnessUnits=N/m  PxLowerLimitDamping=1e3  PxLowerLimitDampingUnits=N/(m/s)  PxLowerLimitTransitionRegionWidth=1e-4  PxLowerLimitTransitionRegionWidthUnits=m  PxUpperLimitSpecify=off  PxUpperLimitBound=1  PxUpperLimitBoundUnits=m  PxUpperLimitStiffness=1e6  PxUpperLimitStiffnessUnits=N/m  PxUpperLimitDamping=1e3  PxUpperLimitDampingUnits=N/(m/s)  PxUpperLimitTransitionRegionWidth=1e-4  PxUpperLimitTransitionRegionWidthUnits=m  PxTorqueActuationMode=ComputedTorque  PxMotionActuationMode=InputMotion  PxSensePosition=on  PxSenseVelocity=off  PxSenseAcceleration=off  PxSenseTorqueForce=on  PxSenseLowerLimitTorqueForce=off  PxSenseUpperLimitTorqueForce=off  PyPositionTargetSpecify=off  PyPositionTargetPriority=High  PyPositionTargetValue=0  PyPositionTargetValueUnits=m  PyVelocityTargetSpecify=off  PyVelocityTargetPriority=High  PyVelocityTargetValue=0  PyVelocityTargetValueUnits=m/s  PyEquilibriumPosition=0  PyEquilibriumPositionUnits=m  PySpringStiffness=0  PySpringStiffnessUnits=N/m  PyDampingCoefficient=0  PyDampingCoefficientUnits=N/(m/s)  PyLowerLimitSpecify=off  PyLowerLimitBound=-1  PyLowerLimitBoundUnits=m  PyLowerLimitStiffness=1e6  PyLowerLimitStiffnessUnits=N/m  PyLowerLimitDamping=1e3  PyLowerLimitDampingUnits=N/(m/s)  PyLowerLimitTransitionRegionWidth=1e-4  PyLowerLimitTransitionRegionWidthUnits=m  PyUpperLimitSpecify=off  PyUpperLimitBound=1  PyUpperLimitBoundUnits=m  PyUpperLimitStiffness=1e6  PyUpperLimitStiffnessUnits=N/m  PyUpperLimitDamping=1e3  PyUpperLimitDampingUnits=N/(m/s)  PyUpperLimitTransitionRegionWidth=1e-4  PyUpperLimitTransitionRegionWidthUnits=m  PyTorqueActuationMode=ComputedTorque  PyMotionActuationMode=InputMotion  PySensePosition=on  PySenseVelocity=off  PySenseAcceleration=off  PySenseTorqueForce=on  PySenseLowerLimitTorqueForce=off  PySenseUpperLimitTorqueForce=off  PzPositionTargetSpecify=off  PzPositionTargetPriority=High  PzPositionTargetValue=0  PzPositionTargetValueUnits=m  PzVelocityTargetSpecify=off  PzVelocityTargetPriority=High  PzVelocityTargetValue=0  PzVelocityTargetValueUnits=m/s  PzEquilibriumPosition=0  PzEquilibriumPositionUnits=m  PzSpringStiffness=0  PzSpringStiffnessUnits=N/m  PzDampingCoefficient=0  PzDampingCoefficientUnits=N/(m/s)  PzLowerLimitSpecify=off  PzLowerLimitBound=-1  PzLowerLimitBoundUnits=m  PzLowerLimitStiffness=1e6  PzLowerLimitStiffnessUnits=N/m  PzLowerLimitDamping=1e3  PzLowerLimitDampingUnits=N/(m/s)  PzLowerLimitTransitionRegionWidth=1e-4  PzLowerLimitTransitionRegionWidthUnits=m  PzUpperLimitSpecify=off  PzUpperLimitBound=1  PzUpperLimitBoundUnits=m  PzUpperLimitStiffness=1e6  PzUpperLimitStiffnessUnits=N/m  PzUpperLimitDamping=1e3  PzUpperLimitDampingUnits=N/(m/s)  PzUpperLimitTransitionRegionWidth=1e-4  PzUpperLimitTransitionRegionWidthUnits=m  PzTorqueActuationMode=ComputedTorque  PzMotionActuationMode=InputMotion  PzSensePosition=on  PzSenseVelocity=off  PzSenseAcceleration=off  PzSenseTorqueForce=on  PzSenseLowerLimitTorqueForce=off  PzSenseUpperLimitTorqueForce=off  SphPositionTargetSpecify=off  SphPositionTargetPriority=High  SphPositionTargetRotationMethod=None  SphPositionTargetFollAlignAxisA=+X  SphPositionTargetBaseAlignAxisA=+Y  SphPositionTargetFollAlignAxisB=+Y  SphPositionTargetBaseAlignAxisB=+Z  SphPositionTargetRotationStandardAxis=+Z  SphPositionTargetRotationAngle=0  SphPositionTargetRotationAngleUnits=deg  SphPositionTargetRotationArbitraryAxis=[0 0 1]  SphPositionTargetRotationSequenceAxes=FollowerAxes  SphPositionTargetRotationSequence=XYX  SphPositionTargetRotationSequenceAngles=[0 0 0]  SphPositionTargetRotationSequenceAnglesUnits=deg  SphPositionTargetRotationMatrix=[1 0 0;0 1 0;0 0 1]  SphPositionTargetQuaternion=[1 0 0 0]  SphVelocityTargetSpecify=off  SphVelocityTargetPriority=High  SphVelocityTargetValue=[0 0 0]  SphVelocityTargetValueUnits=deg/s  SphVelocityTargetInFollowerFrame=on  SphEqPosRotationMethod=None  SphEqPosFollAlignAxisA=+X  SphEqPosBaseAlignAxisA=+Y  SphEqPosFollAlignAxisB=+Y  SphEqPosBaseAlignAxisB=+Z  SphEqPosRotationStandardAxis=+Z  SphEqPosRotationAngle=0  SphEqPosRotationAngleUnits=deg  SphEqPosRotationArbitraryAxis=[0 0 1]  SphEqPosRotationSequenceAxes=FollowerAxes  SphEqPosRotationSequence=XYX  SphEqPosRotationSequenceAngles=[0 0 0]  SphEqPosRotationSequenceAnglesUnits=deg  SphEqPosRotationMatrix=[1 0 0;0 1 0;0 0 1]  SphEqPosQuaternion=[1 0 0 0]  SphSpringStiffness=0  SphSpringStiffnessUnits=N*m/deg  SphDampingCoefficient=0  SphDampingCoefficientUnits=N*m/(deg/s)  SphLowerLimitSpecify=off  SphLowerLimitBound=15  SphLowerLimitBoundUnits=deg  SphLowerLimitStiffness=1e4  SphLowerLimitStiffnessUnits=N*m/deg  SphLowerLimitDamping=10  SphLowerLimitDampingUnits=N*m/(deg/s)  SphLowerLimitTransitionRegionWidth=0.1  SphLowerLimitTransitionRegionWidthUnits=deg  SphUpperLimitSpecify=off  SphUpperLimitBound=45  SphUpperLimitBoundUnits=deg  SphUpperLimitStiffness=1e4  SphUpperLimitStiffnessUnits=N*m/deg  SphUpperLimitDamping=10  SphUpperLimitDampingUnits=N*m/(deg/s)  SphUpperLimitTransitionRegionWidth=0.1  SphUpperLimitTransitionRegionWidthUnits=deg  SphTorqueActuationMode=NoTorque  SphActuateTorqueX=off  SphActuateTorqueY=off  SphActuateTorqueZ=off  SphActuateTorque=off  SphActuationFrame=BaseFrame  SphSensePosition=off  SphSenseVelocityX=off  SphSenseVelocityY=off  SphSenseVelocityZ=off  SphSenseVelocity=off  SphSenseAccelerationX=off  SphSenseAccelerationY=off  SphSenseAccelerationZ=off  SphSenseAcceleration=off  SphSenseLowerLimitTorqueMag=off  SphSenseUpperLimitTorqueMag=off  SphSensingFrame=BaseFrame
  Cartesian Joint : sm_lib/Joints/Cartesian Joint  JointMode=Normal  CompositeWrenchDir=FollowerOnBase  CompositeWrenchFrame=BaseFrame  SenseConstraintForce=off  SenseConstraintTorque=off  SenseTotalForce=off  SenseTotalTorque=off  PxPositionTargetSpecify=off  PxPositionTargetPriority=High  PxPositionTargetValue=0  PxPositionTargetValueUnits=m  PxVelocityTargetSpecify=off  PxVelocityTargetPriority=High  PxVelocityTargetValue=0  PxVelocityTargetValueUnits=m/s  PxEquilibriumPosition=0  PxEquilibriumPositionUnits=m  PxSpringStiffness=0  PxSpringStiffnessUnits=N/m  PxDampingCoefficient=0  PxDampingCoefficientUnits=N/(m/s)  PxLowerLimitSpecify=off  PxLowerLimitBound=-1  PxLowerLimitBoundUnits=m  PxLowerLimitStiffness=1e6  PxLowerLimitStiffnessUnits=N/m  PxLowerLimitDamping=1e3  PxLowerLimitDampingUnits=N/(m/s)  PxLowerLimitTransitionRegionWidth=1e-4  PxLowerLimitTransitionRegionWidthUnits=m  PxUpperLimitSpecify=off  PxUpperLimitBound=1  PxUpperLimitBoundUnits=m  PxUpperLimitStiffness=1e6  PxUpperLimitStiffnessUnits=N/m  PxUpperLimitDamping=1e3  PxUpperLimitDampingUnits=N/(m/s)  PxUpperLimitTransitionRegionWidth=1e-4  PxUpperLimitTransitionRegionWidthUnits=m  PxTorqueActuationMode=ComputedTorque  PxMotionActuationMode=InputMotion  PxSensePosition=on  PxSenseVelocity=off  PxSenseAcceleration=off  PxSenseTorqueForce=off  PxSenseLowerLimitTorqueForce=off  PxSenseUpperLimitTorqueForce=off  PyPositionTargetSpecify=off  PyPositionTargetPriority=High  PyPositionTargetValue=0  PyPositionTargetValueUnits=m  PyVelocityTargetSpecify=off  PyVelocityTargetPriority=High  PyVelocityTargetValue=0  PyVelocityTargetValueUnits=m/s  PyEquilibriumPosition=0  PyEquilibriumPositionUnits=m  PySpringStiffness=0  PySpringStiffnessUnits=N/m  PyDampingCoefficient=0  PyDampingCoefficientUnits=N/(m/s)  PyLowerLimitSpecify=off  PyLowerLimitBound=-1  PyLowerLimitBoundUnits=m  PyLowerLimitStiffness=1e6  PyLowerLimitStiffnessUnits=N/m  PyLowerLimitDamping=1e3  PyLowerLimitDampingUnits=N/(m/s)  PyLowerLimitTransitionRegionWidth=1e-4  PyLowerLimitTransitionRegionWidthUnits=m  PyUpperLimitSpecify=off  PyUpperLimitBound=1  PyUpperLimitBoundUnits=m  PyUpperLimitStiffness=1e6  PyUpperLimitStiffnessUnits=N/m  PyUpperLimitDamping=1e3  PyUpperLimitDampingUnits=N/(m/s)  PyUpperLimitTransitionRegionWidth=1e-4  PyUpperLimitTransitionRegionWidthUnits=m  PyTorqueActuationMode=ComputedTorque  PyMotionActuationMode=InputMotion  PySensePosition=on  PySenseVelocity=off  PySenseAcceleration=off  PySenseTorqueForce=off  PySenseLowerLimitTorqueForce=off  PySenseUpperLimitTorqueForce=off  PzPositionTargetSpecify=off  PzPositionTargetPriority=High  PzPositionTargetValue=0  PzPositionTargetValueUnits=m  PzVelocityTargetSpecify=off  PzVelocityTargetPriority=High  PzVelocityTargetValue=0  PzVelocityTargetValueUnits=m/s  PzEquilibriumPosition=0  PzEquilibriumPositionUnits=m  PzSpringStiffness=0  PzSpringStiffnessUnits=N/m  PzDampingCoefficient=0  PzDampingCoefficientUnits=N/(m/s)  PzLowerLimitSpecify=off  PzLowerLimitBound=-1  PzLowerLimitBoundUnits=m  PzLowerLimitStiffness=1e6  PzLowerLimitStiffnessUnits=N/m  PzLowerLimitDamping=1e3  PzLowerLimitDampingUnits=N/(m/s)  PzLowerLimitTransitionRegionWidth=1e-4  PzLowerLimitTransitionRegionWidthUnits=m  PzUpperLimitSpecify=off  PzUpperLimitBound=1  PzUpperLimitBoundUnits=m  PzUpperLimitStiffness=1e6  PzUpperLimitStiffnessUnits=N/m  PzUpperLimitDamping=1e3  PzUpperLimitDampingUnits=N/(m/s)  PzUpperLimitTransitionRegionWidth=1e-4  PzUpperLimitTransitionRegionWidthUnits=m  PzTorqueActuationMode=ComputedTorque  PzMotionActuationMode=InputMotion  PzSensePosition=on  PzSenseVelocity=off  PzSenseAcceleration=off  PzSenseTorqueForce=off  PzSenseLowerLimitTorqueForce=off  PzSenseUpperLimitTorqueForce=off
  Clock : Clock
  Constant : Constant  Value=trajCoeff
  Constant1 : Constant  Value=trajTime
  MATLAB Function : MATLAB Function  TreatAsAtomicUnit=on
  Mux : Mux  Inputs=3
  PS-Simulink Converter1 : nesl_utility/PS-Simulink Converter  PhysicalDomain=network_engine_domain  SubClassName=ps_output  LeftPortType=input  RightPortType=output  PseudoPeriodic=off  Frequencies=[]  VectorFormat=inherit  Unit=inherit  AffineConversion=off
  PS-Simulink Converter2 : nesl_utility/PS-Simulink Converter  PhysicalDomain=network_engine_domain  SubClassName=ps_output  LeftPortType=input  RightPortType=output  PseudoPeriodic=off  Frequencies=[]  VectorFormat=inherit  Unit=inherit  AffineConversion=off
  PS-Simulink Converter3 : nesl_utility/PS-Simulink Converter  PhysicalDomain=network_engine_domain  SubClassName=ps_output  LeftPortType=input  RightPortType=output  PseudoPeriodic=off  Frequencies=[]  VectorFormat=inherit  Unit=inherit  AffineConversion=off
  Scope1 : Scope  NumInputPorts=3
      settings: ActiveDisplayYMinimum=-0.85197636389002107  ActiveDisplayYMaximum=2.3356362626544458
  Scope2 : Scope  NumInputPorts=3
      settings: ActiveDisplayYMinimum=0.044374041346508353  ActiveDisplayYMaximum=2.4233155506802131  DataLoggingVariableName=ScopeData2
  Simulink-PS Converter : nesl_utility/Simulink-PS Converter  PhysicalDomain=network_engine_domain  SubClassName=ps_input  LeftPortType=input  RightPortType=output  PseudoPeriodic=off  Frequencies=[]  NoiseDistribution=none  NoiseParameters=[]  Unit=1  AffineConversion=off  FilteringAndDerivatives=filter  SimscapeFilterOrder=2  InputFilterTimeConstant=0.001  UdotUserProvided=0
  Simulink-PS Converter1 : nesl_utility/Simulink-PS Converter  PhysicalDomain=network_engine_domain  SubClassName=ps_input  LeftPortType=input  RightPortType=output  PseudoPeriodic=off  Frequencies=[]  NoiseDistribution=none  NoiseParameters=[]  Unit=1  AffineConversion=off  FilteringAndDerivatives=filter  SimscapeFilterOrder=2  InputFilterTimeConstant=0.001  UdotUserProvided=0
  Simulink-PS Converter2 : nesl_utility/Simulink-PS Converter  PhysicalDomain=network_engine_domain  SubClassName=ps_input  LeftPortType=input  RightPortType=output  PseudoPeriodic=off  Frequencies=[]  NoiseDistribution=none  NoiseParameters=[]  Unit=1  AffineConversion=off  FilteringAndDerivatives=filter  SimscapeFilterOrder=2  InputFilterTimeConstant=0.001  UdotUserProvided=0
  World Frame1 : sm_lib/Frames and Transforms/World Frame
  J : PMIOPort  Side=Right
  TCP_Position : Outport
  wires:
  Constant/1 -> MATLAB Function/2(trajCoeff)
  MATLAB Function/2(y) -> Scope1/2, Simulink-PS Converter1/1
  MATLAB Function/3(z) -> Scope1/3, Simulink-PS Converter2/1
  MATLAB Function/1(x) -> Scope1/1, Simulink-PS Converter/1
  Clock/1 -> MATLAB Function/1(t)
  Constant1/1 -> MATLAB Function/3(trajTime)
  Mux/1 -> TCP_Position/1
  PS-Simulink Converter1/1 -> Mux/1, Scope2/1
  PS-Simulink Converter2/1 -> Mux/2, Scope2/2
  PS-Simulink Converter3/1 -> Mux/3, Scope2/3
  connections:
  J/RConn1 -- Cartesian Joint/RConn1
  PS-Simulink Converter2/LConn1 -- Cartesian Joint/RConn3
  Cartesian Joint/LConn1 -- World Frame1/RConn1
  Cartesian Joint/LConn4 -- Simulink-PS Converter2/RConn1
  Cartesian Joint/LConn2 -- Simulink-PS Converter/RConn1
  Cartesian Joint/LConn3 -- Simulink-PS Converter1/RConn1
  PS-Simulink Converter1/LConn1 -- Cartesian Joint/RConn2
  PS-Simulink Converter3/LConn1 -- Cartesian Joint/RConn4
